simulink model "drone"  (R2024a)
settings: Solver=VariableStepAuto  StartTime=0.0  StopTime=5  RelTol=1e-3
values from neighbouring files (symbols this model uses):
  b = 3.13*10^(-5)    (= 3.13e-05)    [drone_p.m]
  d = 7.5*10^(-7)    (= 7.5e-07)    [drone_p.m]
  g = 9.81    [drone_p.m]
  Ir = 6.5*10^(-5)    (= 6.5e-05)    [drone_p.m]
  Ix = 7.5*10^(-3)    (= 0.0075)    [drone_p.m]
  Iy = 7.5*10^(-3)    (= 0.0075)    [drone_p.m]
  Iz = 1.3*10^(-2)    (= 0.013)    [drone_p.m]
  l = 0.23    [drone_p.m]
  m = 0.65    [drone_p.m]
libraries: slpidlib x6
settings Model: SimulationMode=accelerator  Creator=qiu  LastModifiedBy=qiu
settings DataIOCC: ReturnWorkspaceOutputs=off

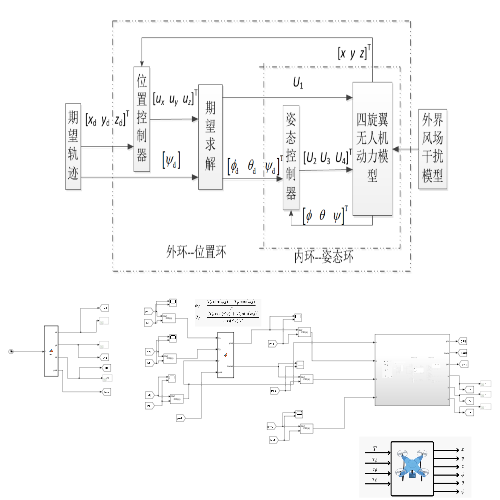
[thumbnail: Simulink's stored preview of the top-level diagram]
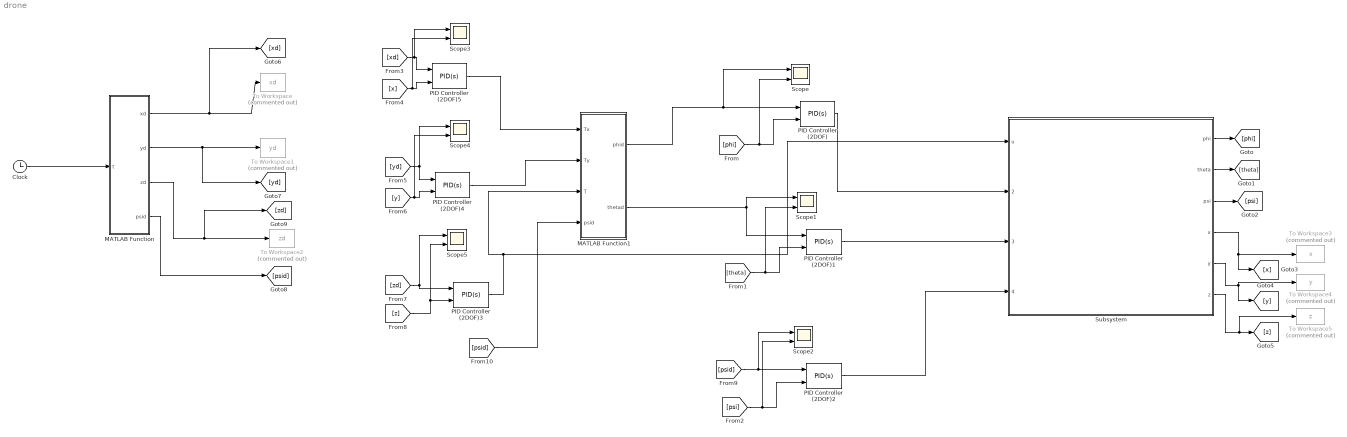
== system drone ==
  Clock : Clock
  MATLAB Function : MATLAB Function  TreatAsAtomicUnit=on
  MATLAB Function1 : MATLAB Function  TreatAsAtomicUnit=on
  PID Controller (2DOF){,1..5} (6 alike) : slpidlib/PID Controller (2DOF)  Controller=PID  Form=Parallel  TimeDomain=Continuous-time  UseExternalTs=off  SampleTime=-1  IntegratorMethod=Forward Euler  FilterMethod=Forward Euler  ControllerParametersSource=internal  P=1  I=1  UseKiTs=off  D=0  UseExternalDerivativeSource=off  N=100  UseFilter=on  b=1  c=1  TunerSelectOption=Transfer Function Based (PID Tuner App)  InitialConditionSource=internal  InitialConditionForIntegrator=0  InitialConditionForFilter=0  DifferentiatorICPrevScaledInput=0  ExternalReset=none  TrackingMode=off  Kt=1  LimitOutput=off  SatLimitsSource=internal  UpperSaturationLimit=inf  LowerSaturationLimit=-inf  LinearizeAsGain=on  AntiWindupMode=none  Kb=1  LimitIntegrator=off  UpperIntegratorSaturationLimit=inf  LowerIntegratorSaturationLimit=-inf  POutMin=[]  POutMax=[]  IOutMin=[]  IOutMax=[]  DOutMin=[]  DOutMax=[]  NOutMin=[]  NOutMax=[]  bOutMin=[]  bOutMax=[]  cOutMin=[]  cOutMax=[]  SumOutMin=[]  SumOutMax=[]  SaturationOutMin=[]  SaturationOutMax=[]  PParamMin=[]  PParamMax=[]  IParamMin=[]  IParamMax=[]  DParamMin=[]  DParamMax=[]  NParamMin=[]  NParamMax=[]  bParamMin=[]  bParamMax=[]  cParamMin=[]  cParamMax=[]  KbParamMin=[]  KbParamMax=[]  KtParamMin=[]  KtParamMax=[]  KbOutMin=[]  KbOutMax=[]  KtOutMin=[]  KtOutMax=[]  IntegratorOutMin=[]  IntegratorOutMax=[]  FilterOutMin=[]  FilterOutMax=[]  SumI1OutMin=[]  SumI1OutMax=[]  SumI2OutMin=[]  SumI2OutMax=[]  SumI3OutMin=[]  SumI3OutMax=[]  SumI4OutMin=[]  SumI4OutMax=[]  SumDOutMin=[]  SumDOutMax=[]  Sum1OutMin=[]  Sum1OutMax=[]  Sum2OutMin=[]  Sum2OutMax=[]  Sum3OutMin=[]  Sum3OutMax=[]  DifferentiatorOutMin=[]  DifferentiatorOutMax=[]  FilterDiffOutCoefMin=[]  FilterDiffOutCoefMax=[]  ReciprocalOutMin=[]  ReciprocalOutMax=[]  SumDenOutMin=[]  SumDenOutMax=[]  SumNumOutMin=[]  SumNumOutMax=[]  DivideOutMin=[]  DivideOutMax=[]  UdiffTsProdOutMin=[]  UdiffTsProdOutMax=[]  NTsProdOutMin=[]  NTsProdOutMax=[]  UintegralTsProdOutMin=[]  UintegralTsProdOutMax=[]  UngainTsProdOutMin=[]  UngainTsProdOutMax=[]  ClampingZeroOutDataTypeStr=Inherit: Inherit via back propagation  ClampingZeroOutMin=[]  ClampingZeroOutMax=[]  FilterDenConstantOutDataTypeStr=Inherit: Inherit via back propagation  FilterDenConstantOutMin=[]  FilterDenConstantOutMax=[]  PCopyOutDataTypeStr=Inherit: Inherit via back propagation  PCopyOutMin=[]  PCopyOutMax=[]  NCopyOutDataTypeStr=Inherit: Inherit via back propagation  NCopyOutMin=[]  NCopyOutMax=[]  IntegratorContinuousStateAttributes=''  IntegratorStateMustResolveToSignalObject=off  IntegratorRTWStateStorageClass=Auto  FilterContinuousStateAttributes=''  FilterStateMustResolveToSignalObject=off  FilterRTWStateStorageClass=Auto  ParallelPVariant=InternalParameters  IdealPVariant=Disabled  IVariant=InternalParameters  DVariant=InternalParameters  bVariant=InternalParameters  cVariant=InternalParameters  IntegratorVariant=Continuous  SatVariant=Disabled  AWVariant=Passthrough  PCopyVariant=Disabled  TRVariant=Disabled  FdbkBlocksVariant=Forward  IdealPFdbkVariant=Disabled  SatFdbkVariant=Disabled  DerivativeFilterVariant=ContFilter  NVariant=InternalParameters  NCopyVariant=Disabled  FilterICVariant=InternalICsFilter  IntegratorICVariant=InternalICs  ExternalResetVariant=Disabled  TRSumVariant=Passthrough  SumFdbkVariant=Disabled  SumVariant=Sum_PID  TsampFilterVariant=InternalTs  TsampNgainVariant=Passthrough  TsampIntegralVariant=Disabled_SignalSpec  ExternalSaturationOutDataTypeStr=Inherit: Same as second input  DerivativeSourceVariant=ErrorSignal
  Scope{,1..5} (6 alike) : Scope  NumInputPorts=2
  Subsystem : Subsystem
  To Workspace : ToWorkspace  Commented=on  VariableName=xd  SampleTime=-1
  To Workspace1 : ToWorkspace  Commented=on  VariableName=yd  SampleTime=-1
  To Workspace2 : ToWorkspace  Commented=on  VariableName=zd  SampleTime=-1
  To Workspace3 : ToWorkspace  Commented=on  VariableName=x  SampleTime=-1
  To Workspace4 : ToWorkspace  Commented=on  VariableName=y  SampleTime=-1
  To Workspace5 : ToWorkspace  Commented=on  VariableName=z  SampleTime=-1
  wires:
  Subsystem/1(phi) -> [phi]
  Subsystem/2(theta) -> [theta]
  Subsystem/3(psi) -> [psi]
  [phi] -> PID Controller (2DOF)/2, Scope/2
  PID Controller (2DOF)/1 -> Subsystem/2(2)
  MATLAB Function1/2(thetad) -> PID Controller (2DOF)1/1, Scope1/1
  PID Controller (2DOF)1/1 -> Subsystem/3(3)
  [theta] -> PID Controller (2DOF)1/2, Scope1/2
  [psi] -> PID Controller (2DOF)2/2, Scope2/2
  [psid] -> PID Controller (2DOF)2/1, Scope2/1
  PID Controller (2DOF)2/1 -> Subsystem/4(4)
  Clock/1 -> MATLAB Function/1(t)
  MATLAB Function/1(xd) -> [xd], To Workspace/1
  MATLAB Function/2(yd) -> [yd], To Workspace1/1
  MATLAB Function/3(zd) -> [zd], To Workspace2/1
  Subsystem/4(x) -> [x], To Workspace3/1
  Subsystem/5(y) -> [y], To Workspace4/1
  Subsystem/6(z) -> To Workspace5/1, [z]
  [xd] -> PID Controller (2DOF)5/1, Scope3/1
  [x] -> PID Controller (2DOF)5/2, Scope3/2
  [yd] -> PID Controller (2DOF)4/1, Scope4/1
  [y] -> PID Controller (2DOF)4/2, Scope4/2
  [zd] -> PID Controller (2DOF)3/1, Scope5/1
  [z] -> PID Controller (2DOF)3/2, Scope5/2
  PID Controller (2DOF)5/1 -> MATLAB Function1/1(Tx)
  PID Controller (2DOF)4/1 -> MATLAB Function1/2(Ty)
  PID Controller (2DOF)3/1 -> MATLAB Function1/3(T), Subsystem/1(u)
  [psid] -> MATLAB Function1/4(psid)
  MATLAB Function/4(psid) -> [psid]
  MATLAB Function1/1(phid) -> PID Controller (2DOF)/1, Scope/1

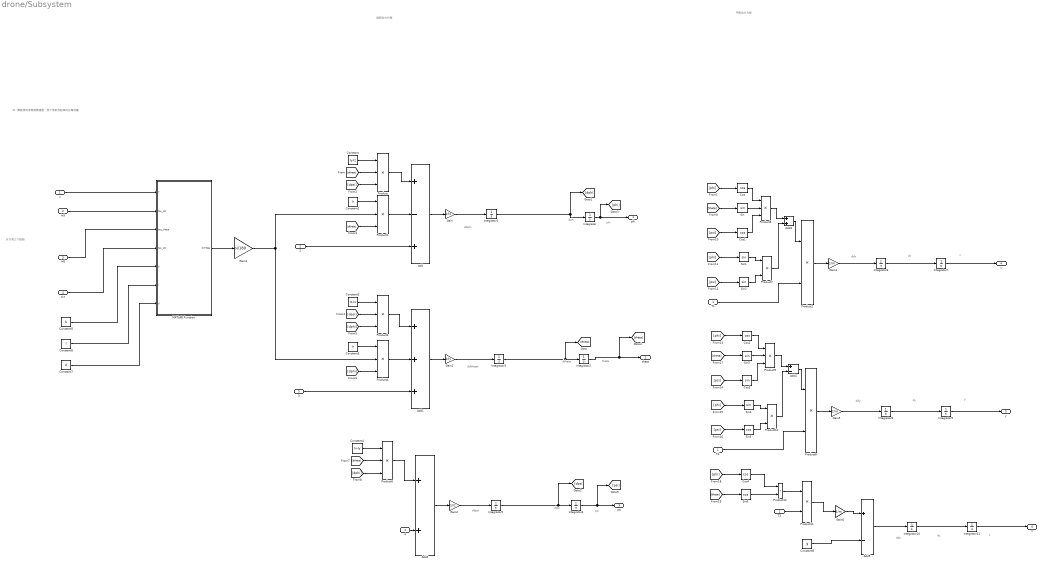
== system drone/Subsystem ==
  note: Ω：螺旋桨的净自旋角速度，四个电机合起来的总角动量
  note: 升力和三个扭矩
  note: 旋转动力方程
  note: ddx
  note: ddphi
  note: dphi
  note: phi
  note: dtheta
  note: ddthetai
  note: theta
  note: dpsi
  note: ddpsi
  note: psi
  note: x
  note: dx
  note: y
  note: dy
  note: ddy
  note: z
  note: dz
  note: ddz
  note: 平移动力方程
  u : Inport
  2 : Inport  Port=2
  3 : Inport  Port=3
  4 : Inport  Port=4
  Add : Sum  Inputs=+-+
  Add1 : Sum  Inputs=+++
  Add2 : Sum
  Add3 : Sum
  Add4 : Sum  Inputs=+-
  Add5 : Sum  Inputs=+-
  Constant : Constant  Value=Iy-Iz
  Constant1 : Constant  Value=Ir
  Constant2 : Constant  Value=Iz-Ix
  Constant3 : Constant  Value=Ir
  Constant4 : Constant  Value=Ix-Iy
  Constant5 : Constant  Value=b
  Constant6 : Constant  Value=l
  Constant7 : Constant  Value=d
  Constant8 : Constant  Value=g
  Cos{,1..2,4} (4 alike) : Trigonometry  Operator=cos
  Cos3 : Trigonometry
  Gain : Gain  Gain=1/Ix
  Gain1 : Gain  Gain=1/Iy
  Gain2 : Gain  Gain=1/Iz
  Gain3 : Gain  Gain=pi/180
  Gain4 : Gain  Gain=1/m
  Gain5 : Gain  Gain=1/m
  Gain6 : Gain  Gain=1/m
  In5 : InportShadow  Port=2
  In6 : InportShadow  Port=3
  In7 : InportShadow  Port=4
  Integrator{,1..11} (12 alike) : Integrator
  MATLAB Function : MATLAB Function  TreatAsAtomicUnit=on
  Product{,1,3..7,9..10} (9 alike) : Product  Inputs=3
  Product{2,8,11..12} (4 alike) : Product
  Sin{,1..4} (5 alike) : Trigonometry
  Sin5 : Trigonometry  Operator=cos
  Sin6 : Trigonometry  Operator=cos
  T1 : InportShadow
  T3 : InportShadow
  T4 : InportShadow
  phi : Outport
  theta : Outport  Port=2
  psi : Outport  Port=3
  x : Outport  Port=4
  y : Outport  Port=5
  z : Outport  Port=6
  wires:
  [dtheta] -> Product1/3
  4/1 -> Add2/2
  [dphi] -> Product3/3
  Integrator4/1 -> [psi], psi/1
  Gain/1 -> Integrator1/1
  Gain2/1 -> Integrator5/1
  Integrator5/1 -> [dpsi], Integrator4/1
  [dpsi] -> Product3/2
  Integrator3/1 -> [dtheta], Integrator2/1
  Constant3/1 -> Product4/1
  Constant2/1 -> Product3/1
  [dpsi] -> Product/3
  Add1/1 -> Gain1/1
  MATLAB Function/1(Omega) -> Gain3/1
  Add/1 -> Gain/1
  [dtheta] -> Product6/2
  [dphi] -> Product4/3
  2/1 -> Add/3
  Product3/1 -> Add1/1
  Constant1/1 -> Product1/1
  Integrator2/1 -> [theta], theta/1
  Integrator1/1 -> Integrator/1, [dphi]
  Constant/1 -> Product/1
  Constant4/1 -> Product6/1
  Gain1/1 -> Integrator3/1
  [dphi] -> Product6/3
  Product6/1 -> Add2/1
  Add2/1 -> Gain2/1
  Integrator/1 -> [phi], phi/1
  Product4/1 -> Add1/2
  Product/1 -> Add/1
  [dtheta] -> Product/2
  Product1/1 -> Add/2
  3/1 -> Add1/3
  u/1 -> MATLAB Function/1(T)
  In5/1 -> MATLAB Function/2(tau_phi)
  In6/1 -> MATLAB Function/3(tau_theta)
  In7/1 -> MATLAB Function/4(tau_psi)
  Constant5/1 -> MATLAB Function/5(b)
  Constant6/1 -> MATLAB Function/6(l)
  Constant7/1 -> MATLAB Function/7(d)
  Gain3/1 -> Product1/2, Product4/2
  Integrator6/1 -> Integrator7/1
  Integrator7/1 -> x/1
  Gain4/1 -> Integrator6/1
  Gain5/1 -> Integrator8/1
  Integrator8/1 -> Integrator9/1
  Integrator9/1 -> y/1
  Add5/1 -> Integrator10/1
  Integrator10/1 -> Integrator11/1
  Integrator11/1 -> z/1
  Product2/1 -> Gain4/1
  Add3/1 -> Product2/1
  [psi] -> Cos1/1
  [theta] -> Sin/1
  [phi] -> Cos/1
  Cos/1 -> Product5/1
  Sin/1 -> Product5/2
  Cos1/1 -> Product5/3
  Product5/1 -> Add3/1
  [phi] -> Sin1/1
  [psi] -> Sin2/1
  Sin1/1 -> Product7/1
  Sin2/1 -> Product7/3
  Product7/1 -> Add3/2
  T1/1 -> Product2/2
  [theta] -> Sin3/1
  Sin3/1 -> Product9/2
  Cos3/1 -> Product9/3
  [psi] -> Sin5/1
  [phi] -> Sin4/1
  Cos2/1 -> Product9/1
  Add4/1 -> Product8/1
  Product8/1 -> Gain5/1
  Product9/1 -> Add4/1
  Sin4/1 -> Product10/1
  [phi] -> Cos2/1
  [psi] -> Cos3/1
  Sin5/1 -> Product10/3
  Product10/1 -> Add4/2
  T4/1 -> Product8/2
  Constant8/1 -> Add5/2
  Product11/1 -> Gain6/1
  T3/1 -> Product11/2
  Product12/1 -> Product11/1
  [theta] -> Sin6/1
  [phi] -> Cos4/1
  Cos4/1 -> Product12/1
  Sin6/1 -> Product12/2
  Gain6/1 -> Add5/1

== matlab function drone/MATLAB Function ==
  data: t input; xd output; yd output; zd output; psid output
function [xd,yd,zd,psid] = fcn(t)
xd = cos(0.2*t);
yd = sin(0.2*t);
zd = 10*t;
psid = sin(t);

== matlab function drone/Subsystem/MATLAB Function ==
  data: T input; Omega output; tau_phi input; tau_theta input; tau_psi input; b input; l input; d input
function Omega = fcn(T,tau_phi, tau_theta,tau_psi, b, l, d)

U1 = T/b;
U2 = tau_phi/l*b;
U3 = tau_theta/l*b;
U4 = tau_psi/d;

omega_3 = sqrt(max(0, (U1 + U4 + 2*U2)/4));

omega_1 = sqrt(max(0, (U1 + U4 - 2*U2)/4));

omega_4 = sqrt(max(0, (U1 - U4 + 2*U3)/4));

omega_2 = sqrt(max(0, (U1 - U4 - 2*U3)/4));

Omega = omega_1 - omega_2 + omega_3 - omega_4;

== matlab function drone/MATLAB Function1 ==
  data: Tx input; phid output; Ty input; T input; psid input; thetad output
function [phid,thetad] = fcn(Tx, Ty,T, psid)

phid = (Tx*sin(psid) - Ty*cos(psid))/T;
thetad = ((Tx*cos(psid) + Ty*sin(psid))/cos(phid))/T;

phid = max(phid,-pi/6);
phid = min(phid,pi/6);

thetad = max(thetad, -pi/6);
thetad = min(thetad, pi/6);
